simulink model "sst_cllc_ttype_inv_discrete"  (R2026b)
settings: Solver=ode23tb  StopTime=simlength  FixedStep=tc  MaxStep=glb_time.tc
values from neighbouring files (symbols this model uses):
  param = sst_cllc_ttype_setup(param)    [init_model.m]
undefined symbols (not defined in the file or in its folder): afe_ctrl, glb_time, grid_emu, hwdata, omega_set, single_phase_inverter_ctrl, sst_num_of_modules
libraries: fl_lib x28, nesl_utility x16, discrete_time_low_pass_filter x4, lithium_ion_battery x2, cllc_dcx x2, dclink_for_three_levels x2, full_bridge_three_level_ttype_ideal_switch_based_model x2, full_bridge_three_level_ttype_mosfet_based_model x2, simulink x2, cstblocks_lti x2, single_phase_three_levels_PWM_modulator x2, dq_vector_pi x2
(part 3 of 3)

== system sst_cllc_ttype_inv_discrete/single_phase_inverter_modA/single phase inverter control/single_phase_inverter_ctrl/single_phase_pll/pi-ctrl ==
  x : Inport
  xref : Inport  Port=2
  1/Ti : Gain  Gain=kp  SaturateOnIntegerOverflow=on  OutDataTypeStr=Inherit: Same as input  ParamDataTypeStr=Inherit: Same as input
  Saturation : Saturate  UpperLimit=sat_pos  LowerLimit=sat_neg
  Sum1 : Sum  Inputs=+++  SaturateOnIntegerOverflow=on
  Sum2 : Sum  Inputs=-+  SaturateOnIntegerOverflow=on
  Sum3 : Sum  Inputs=-+  SaturateOnIntegerOverflow=on
  Unit Delay4 : UnitDelay  SampleTime=-1
  kp : Gain  Gain=ki*ts  SaturateOnIntegerOverflow=on  OutDataTypeStr=Inherit: Same as input  ParamDataTypeStr=Inherit: Same as input
  u : Outport
  wires:
  Saturation/1 -> Sum3/2, u/1
  Unit Delay4/1 -> Sum1/3
  Sum1/1 -> Saturation/1
  Sum3/1 -> Unit Delay4/1
  1/Ti/1 -> Sum3/1, Sum1/1
  Sum2/1 -> 1/Ti/1, kp/1
  kp/1 -> Sum1/2
  x/1 -> Sum2/1
  xref/1 -> Sum2/2

== system sst_cllc_ttype_inv_discrete/single_phase_inverter_modB/single phase inverter control/single_phase_inverter_ctrl/single_phase_current_control/current_reference_generation ==
  mag_ref : Inport
  phase : Inport  Port=2
  Bus Creator : BusCreator  Inputs=2
  Product : Product
  Product1 : Product
  Sin : Trigonometry  Operator=cos
  Sin1 : Trigonometry
  is_ref : Outport
  id_ref : Outport  Port=2
  wires:
  Bus Creator/1 -> is_ref/1
  Product1/1 -> Bus Creator/2  "is_ref_beta"
  Product/1 -> Bus Creator/1  "is_ref_alpha"
  Sin1/1 -> Product1/2
  mag_ref/1 -> Product/1, Product1/1, id_ref/1
  phase/1 -> Sin/1, Sin1/1
  Sin/1 -> Product/2

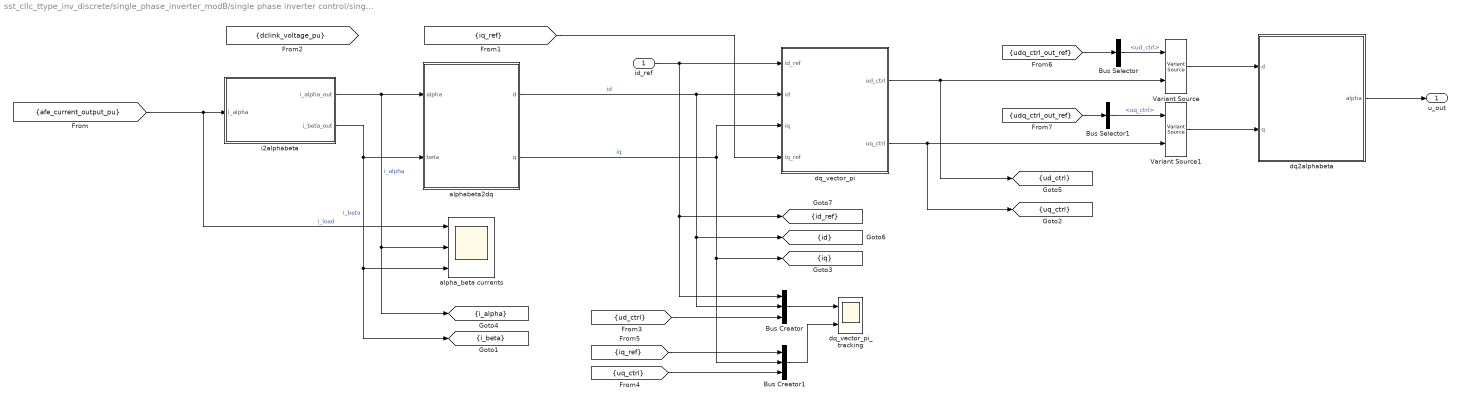
== system sst_cllc_ttype_inv_discrete/single_phase_inverter_modB/single phase inverter control/single_phase_inverter_ctrl/single_phase_current_control/dqpi_current_controller ==
  id_ref : Inport
  Bus Creator : BusCreator  Inputs=3
  Bus Creator1 : BusCreator  Inputs=3
  Bus Selector : BusSelector  OutputSignals=ud_ctrl
  Bus Selector1 : BusSelector  OutputSignals=uq_ctrl
  Variant Source : VariantSource  VariantControls={true, false}
  Variant Source1 : VariantSource  VariantControls={true, false}
  alpha_beta currents : Scope  NumInputPorts=3
      settings: ActiveDisplayYMinimum=-43.020049026506776  ActiveDisplayYMaximum=15.212667801061009  DataLoggingVariableName=ScopeData2
  alphabeta2dq : Subsystem
  dq2alphabeta : Subsystem
  dq_vector_pi : Subsystem
  dq_vector_pi_tracking : Scope  NumInputPorts=2
      settings: ActiveDisplayYMinimum=-5.8450231123834442  ActiveDisplayYMaximum=20.947282871449747  DataLoggingVariableName=ScopeData8
  i2alphabeta : Subsystem
  u_out : Outport
  tag scope: i_alpha=scoped, i_beta=scoped, id=scoped, id_ref=scoped, iq=scoped, ud_ctrl=scoped, uq_ctrl=scoped
  wires:
  dq_vector_pi/1(ud_ctrl) -> [ud_ctrl], Variant Source/2
  i2alphabeta/2(i_beta_out) -> alphabeta2dq/2(beta), alpha_beta currents/3, [i_beta]  "i_beta"
  i2alphabeta/1(i_alpha_out) -> alphabeta2dq/1(alpha), [i_alpha], alpha_beta currents/2  "i_alpha"
  [afe_current_output_pu] -> i2alphabeta/1(i_alpha), alpha_beta currents/1  "i_load"
  [iq_ref] -> Bus Creator1/1
  [uq_ctrl] -> Bus Creator1/3
  [ud_ctrl] -> Bus Creator/3
  Bus Creator/1 -> dq_vector_pi_tracking/1
  Bus Creator1/1 -> dq_vector_pi_tracking/2
  [iq_ref] -> dq_vector_pi/4(iq_ref)
  alphabeta2dq/2("q ") -> [iq], Bus Creator1/2, dq_vector_pi/3(iq)  "iq"
  alphabeta2dq/1("d ") -> dq_vector_pi/2(id), [id], Bus Creator/2  "id"
  id_ref/1 -> [id_ref], Bus Creator/1, dq_vector_pi/1(id_ref)
  dq2alphabeta/1(alpha) -> u_out/1
  [udq_ctrl_out_ref] -> Bus Selector/1
  Variant Source/1 -> dq2alphabeta/1(d)
  Bus Selector/1 -> Variant Source/1  "<ud_ctrl>"
  Bus Selector1/1 -> Variant Source1/1  "<uq_ctrl>"
  [udq_ctrl_out_ref] -> Bus Selector1/1
  dq_vector_pi/2(uq_ctrl) -> Variant Source1/2, [uq_ctrl]
  Variant Source1/1 -> dq2alphabeta/2(q)

== system sst_cllc_ttype_inv_discrete/single_phase_inverter_modB/single phase inverter control/single_phase_inverter_ctrl/single_phase_pll/double_integrator_observer ==
  theta : Inport
  Gain : Gain  Gain=afe_ctrl.di_obs.Ldso  Multiplication=Matrix(K*u)
  Gain1 : Gain  Gain=afe_ctrl.di_obs.Adso  Multiplication=Matrix(K*u)
  Gain2 : Gain  Gain=afe_ctrl.di_obs.Cso  Multiplication=Matrix(K*u)
  Selector : Selector  InputPortWidth=2  IndexOptions=Index vector (dialog)  Indices=2  OutputSizes=1  RuntimeRangeChecks=off
  Sum : Sum  Inputs=-+|
  Sum1 : Sum  Inputs=|++
  Unit Delay : UnitDelay  SampleTime=-1
  bounder1 : MATLAB Function  TreatAsAtomicUnit=on
  bounder2 : MATLAB Function  TreatAsAtomicUnit=on
  kp3 : Gain  Gain=1/grid_emu.omega_grid_nom  SaturateOnIntegerOverflow=on  OutDataTypeStr=Inherit: Same as input  ParamDataTypeStr=Inherit: Same as input
  phase_hat : Outport
  omega_hat : Outport  Port=2
  wires:
  kp3/1 -> omega_hat/1
  Selector/1 -> kp3/1
  bounder2/1(y) -> Sum/1, phase_hat/1  "theta_hat_bounded"
  bounder1/1(y) -> Gain/1  "e_bounded"
  theta/1 -> Sum/2  "theta"
  Unit Delay/1 -> Gain2/1, Gain1/1, Selector/1
  Sum/1 -> bounder1/1(u)  "e"
  Sum1/1 -> Unit Delay/1
  Gain1/1 -> Sum1/2
  Gain2/1 -> bounder2/1(u)  "theta_hat"
  Gain/1 -> Sum1/1

== system sst_cllc_ttype_inv_discrete/single_phase_inverter_modB/single phase inverter control/single_phase_inverter_ctrl/single_phase_pll/pi-ctrl ==
  x : Inport
  xref : Inport  Port=2
  1/Ti : Gain  Gain=kp  SaturateOnIntegerOverflow=on  OutDataTypeStr=Inherit: Same as input  ParamDataTypeStr=Inherit: Same as input
  Saturation : Saturate  UpperLimit=sat_pos  LowerLimit=sat_neg
  Sum1 : Sum  Inputs=+++  SaturateOnIntegerOverflow=on
  Sum2 : Sum  Inputs=-+  SaturateOnIntegerOverflow=on
  Sum3 : Sum  Inputs=-+  SaturateOnIntegerOverflow=on
  Unit Delay4 : UnitDelay  SampleTime=-1
  kp : Gain  Gain=ki*ts  SaturateOnIntegerOverflow=on  OutDataTypeStr=Inherit: Same as input  ParamDataTypeStr=Inherit: Same as input
  u : Outport
  wires:
  xref/1 -> Sum2/2
  x/1 -> Sum2/1
  kp/1 -> Sum1/2
  Sum2/1 -> kp/1, 1/Ti/1
  1/Ti/1 -> Sum1/1, Sum3/1
  Sum3/1 -> Unit Delay4/1
  Sum1/1 -> Saturation/1
  Unit Delay4/1 -> Sum1/3
  Saturation/1 -> u/1, Sum3/2

== system sst_cllc_ttype_inv_discrete/single_phase_inverter_modA/single phase inverter control/single_phase_inverter_ctrl/single_phase_current_control/dqpi_current_controller/alphabeta2dq ==
  alpha : Inport
  beta : Inport  Port=2
  MATLAB Function : MATLAB Function  TreatAsAtomicUnit=on
  "d " : Outport  VectorParamsAs1DForOutWhenUnconnected=off
  "q " : Outport  Port=2  VectorParamsAs1DForOutWhenUnconnected=off
  wires:
  alpha/1 -> MATLAB Function/1(alpha)
  beta/1 -> MATLAB Function/2(beta)
  MATLAB Function/1(d) -> "d "/1
  MATLAB Function/2(q) -> "q "/1
  [phase_grid] -> MATLAB Function/3(phase)

== system sst_cllc_ttype_inv_discrete/single_phase_inverter_modA/single phase inverter control/single_phase_inverter_ctrl/single_phase_current_control/dqpi_current_controller/dq2alphabeta ==
  d : Inport
  q : Inport  Port=2
  MATLAB Function : MATLAB Function  TreatAsAtomicUnit=on
  alpha : Outport  VectorParamsAs1DForOutWhenUnconnected=off
  wires:
  d/1 -> MATLAB Function/1(d)
  q/1 -> MATLAB Function/2(q)
  MATLAB Function/1(alpha) -> alpha/1
  [phase_grid] -> MATLAB Function/3(phase)

== system sst_cllc_ttype_inv_discrete/single_phase_inverter_modA/single phase inverter control/single_phase_inverter_ctrl/single_phase_current_control/dqpi_current_controller/dq_vector_pi ==
  id_ref : Inport
  id : Inport  Port=2
  iq : Inport  Port=3
  iq_ref : Inport  Port=4
  dq_vector_pi : dq_vector_pi/dq_vector_pi  kp=single_phase_inverter_ctrl.kp_inv  ki=single_phase_inverter_ctrl.ki_inv  ts=glb_time.ts_inv  lim_ctrl_out=single_phase_inverter_ctrl.u_lim  CTRPIFF_CLIP_RELEASE=CTRPIFF_CLIP_RELEASE
  ud_ctrl : Outport
  uq_ctrl : Outport  Port=2
  wires:
  id_ref/1 -> dq_vector_pi/1  "id_ref"
  iq_ref/1 -> dq_vector_pi/3  "iq_ref"
  dq_vector_pi/1 -> ud_ctrl/1  "ud_ctrl"
  iq/1 -> dq_vector_pi/4  "iq"
  id/1 -> dq_vector_pi/2  "id"
  dq_vector_pi/2 -> uq_ctrl/1  "uq_ctrl"
  [dclink_voltage_pu] -> dq_vector_pi/5

== system sst_cllc_ttype_inv_discrete/single_phase_inverter_modA/single phase inverter control/single_phase_inverter_ctrl/single_phase_current_control/dqpi_current_controller/i2alphabeta ==
  i_alpha : Inport
  FHTalpha : Subsystem
  i_alpha_out : Outport
  i_beta_out : Outport  Port=2
  wires:
  i_alpha/1 -> FHTalpha/1(u)
  FHTalpha/1(ualpha) -> i_alpha_out/1  "u_fht_alpha"
  FHTalpha/2(ubeta) -> i_beta_out/1  "v_fht_alpha"

== system sst_cllc_ttype_inv_discrete/single_phase_inverter_modB/single phase inverter control/single_phase_inverter_ctrl/single_phase_current_control/dqpi_current_controller/alphabeta2dq ==
  alpha : Inport
  beta : Inport  Port=2
  MATLAB Function : MATLAB Function  TreatAsAtomicUnit=on
  "d " : Outport  VectorParamsAs1DForOutWhenUnconnected=off
  "q " : Outport  Port=2  VectorParamsAs1DForOutWhenUnconnected=off
  wires:
  [phase_grid] -> MATLAB Function/3(phase)
  MATLAB Function/2(q) -> "q "/1
  MATLAB Function/1(d) -> "d "/1
  beta/1 -> MATLAB Function/2(beta)
  alpha/1 -> MATLAB Function/1(alpha)

== system sst_cllc_ttype_inv_discrete/single_phase_inverter_modB/single phase inverter control/single_phase_inverter_ctrl/single_phase_current_control/dqpi_current_controller/dq2alphabeta ==
  d : Inport
  q : Inport  Port=2
  MATLAB Function : MATLAB Function  TreatAsAtomicUnit=on
  alpha : Outport  VectorParamsAs1DForOutWhenUnconnected=off
  wires:
  [phase_grid] -> MATLAB Function/3(phase)
  MATLAB Function/1(alpha) -> alpha/1
  q/1 -> MATLAB Function/2(q)
  d/1 -> MATLAB Function/1(d)

== system sst_cllc_ttype_inv_discrete/single_phase_inverter_modB/single phase inverter control/single_phase_inverter_ctrl/single_phase_current_control/dqpi_current_controller/dq_vector_pi ==
  id_ref : Inport
  id : Inport  Port=2
  iq : Inport  Port=3
  iq_ref : Inport  Port=4
  dq_vector_pi : dq_vector_pi/dq_vector_pi  kp=single_phase_inverter_ctrl.kp_inv  ki=single_phase_inverter_ctrl.ki_inv  ts=glb_time.ts_inv  lim_ctrl_out=single_phase_inverter_ctrl.u_lim  CTRPIFF_CLIP_RELEASE=CTRPIFF_CLIP_RELEASE
  ud_ctrl : Outport
  uq_ctrl : Outport  Port=2
  wires:
  [dclink_voltage_pu] -> dq_vector_pi/5
  dq_vector_pi/2 -> uq_ctrl/1  "uq_ctrl"
  id/1 -> dq_vector_pi/2  "id"
  iq/1 -> dq_vector_pi/4  "iq"
  dq_vector_pi/1 -> ud_ctrl/1  "ud_ctrl"
  iq_ref/1 -> dq_vector_pi/3  "iq_ref"
  id_ref/1 -> dq_vector_pi/1  "id_ref"

== system sst_cllc_ttype_inv_discrete/single_phase_inverter_modB/single phase inverter control/single_phase_inverter_ctrl/single_phase_current_control/dqpi_current_controller/i2alphabeta ==
  i_alpha : Inport
  FHTalpha : Subsystem
  i_alpha_out : Outport
  i_beta_out : Outport  Port=2
  wires:
  FHTalpha/2(ubeta) -> i_beta_out/1  "v_fht_alpha"
  FHTalpha/1(ualpha) -> i_alpha_out/1  "u_fht_alpha"
  i_alpha/1 -> FHTalpha/1(u)

== system sst_cllc_ttype_inv_discrete/single_phase_inverter_modA/single phase inverter control/single_phase_inverter_ctrl/single_phase_current_control/dqpi_current_controller/i2alphabeta/FHTalpha ==
  u : Inport
  Gain : Gain  Gain=single_phase_inverter_ctrl.fht_load.Ld_fht  Multiplication=Matrix(K*u)
  Gain1 : Gain  Gain=single_phase_inverter_ctrl.fht_load.Ad_fht  Multiplication=Matrix(K*u)
  Gain2 : Gain  Gain=single_phase_inverter_ctrl.fht_load.Cfht  Multiplication=Matrix(K*u)
  Gain3 : Gain  Gain=-1/single_phase_inverter_ctrl.omega_base
  Selector : Selector  InputPortWidth=2  IndexOptions=Index vector (dialog)  Indices=1  OutputSizes=1  RuntimeRangeChecks=off
  Selector1 : Selector  InputPortWidth=2  IndexOptions=Index vector (dialog)  Indices=2  OutputSizes=1  RuntimeRangeChecks=off
  Sum : Sum  Inputs=-+|
  Sum1 : Sum  Inputs=|++
  Unit Delay : UnitDelay  SampleTime=-1
  ualpha : Outport
  ubeta : Outport  Port=2
  wires:
  u/1 -> Sum/2
  Unit Delay/1 -> Gain2/1, Selector1/1, Selector/1, Gain1/1
  Sum/1 -> Gain/1
  Sum1/1 -> Unit Delay/1
  Gain1/1 -> Sum1/2
  Gain2/1 -> Sum/1
  Selector/1 -> ualpha/1
  Gain/1 -> Sum1/1
  Selector1/1 -> Gain3/1
  Gain3/1 -> ubeta/1

== system sst_cllc_ttype_inv_discrete/single_phase_inverter_modB/single phase inverter control/single_phase_inverter_ctrl/single_phase_current_control/dqpi_current_controller/i2alphabeta/FHTalpha ==
  u : Inport
  Gain : Gain  Gain=single_phase_inverter_ctrl.fht_load.Ld_fht  Multiplication=Matrix(K*u)
  Gain1 : Gain  Gain=single_phase_inverter_ctrl.fht_load.Ad_fht  Multiplication=Matrix(K*u)
  Gain2 : Gain  Gain=single_phase_inverter_ctrl.fht_load.Cfht  Multiplication=Matrix(K*u)
  Gain3 : Gain  Gain=-1/single_phase_inverter_ctrl.omega_base
  Selector : Selector  InputPortWidth=2  IndexOptions=Index vector (dialog)  Indices=1  OutputSizes=1  RuntimeRangeChecks=off
  Selector1 : Selector  InputPortWidth=2  IndexOptions=Index vector (dialog)  Indices=2  OutputSizes=1  RuntimeRangeChecks=off
  Sum : Sum  Inputs=-+|
  Sum1 : Sum  Inputs=|++
  Unit Delay : UnitDelay  SampleTime=-1
  ualpha : Outport
  ubeta : Outport  Port=2
  wires:
  Gain3/1 -> ubeta/1
  Selector1/1 -> Gain3/1
  Gain/1 -> Sum1/1
  Selector/1 -> ualpha/1
  Gain2/1 -> Sum/1
  Gain1/1 -> Sum1/2
  Sum1/1 -> Unit Delay/1
  Sum/1 -> Gain/1
  Unit Delay/1 -> Gain1/1, Selector/1, Selector1/1, Gain2/1
  u/1 -> Sum/2

== matlab function sst_cllc_ttype_inv_discrete/single_phase_inverter_modB/single phase inverter control/single_phase_inverter_ctrl/single_phase_pll/alphabeta2xieta ==
  data: alpha input; xi output; beta input; gamma input; eta output
function [xi,eta] = alphabeta2xieta(alpha,beta,gamma)
    xi  =  alpha*cos(gamma) + beta*sin(gamma);
    eta = -alpha*sin(gamma) + beta*cos(gamma);
end

== matlab function sst_cllc_ttype_inv_discrete/single_phase_inverter_modB/single phase inverter control/single_phase_inverter_ctrl/single_phase_pll/bounder2 ==
  data: u input; y output
function y = bounder(u)
    
    y = -pi + mod(u+3*pi,2*pi);
   
end

== matlab function sst_cllc_ttype_inv_discrete/single_phase_inverter_modB/single phase inverter control/single_phase_inverter_ctrl/single_phase_pll/double_integrator_observer/bounder1 ==
  data: u input; y output
function y = bounder(u)
    
    y = -pi + mod(u+3*pi,2*pi);
   
end

== matlab function sst_cllc_ttype_inv_discrete/single_phase_inverter_modB/single phase inverter control/single_phase_inverter_ctrl/single_phase_pll/double_integrator_observer/bounder2 ==
  data: u input; y output
function y = bounder(u)
    
    y = -pi + mod(u+3*pi,2*pi);
   
end

== matlab function sst_cllc_ttype_inv_discrete/single_phase_inverter_modB/single phase inverter control/single_phase_inverter_ctrl/single_phase_pll/xieta2alphabeta ==
  data: xi input; alpha output; eta input; gamma input; beta output
function [alpha,beta] = xieta2alphabeta(xi,eta,gamma)
    alpha  = xi*cos(gamma) - eta*sin(gamma);
    beta = xi*sin(gamma) + eta*cos(gamma);
end

== matlab function sst_cllc_ttype_inv_discrete/single_phase_inverter_modA/single phase inverter control/single_phase_inverter_ctrl/single_phase_pll/double_integrator_observer/bounder1 ==
  data: u input; y output
function y = bounder(u)
    
    y = -pi + mod(u+3*pi,2*pi);
   
end

== matlab function sst_cllc_ttype_inv_discrete/single_phase_inverter_modA/single phase inverter control/single_phase_inverter_ctrl/single_phase_pll/double_integrator_observer/bounder2 ==
  data: u input; y output
function y = bounder(u)
    
    y = -pi + mod(u+3*pi,2*pi);
   
end

== matlab function sst_cllc_ttype_inv_discrete/single_phase_inverter_modA/single phase inverter control/single_phase_inverter_ctrl/single_phase_pll/xieta2alphabeta ==
  data: xi input; alpha output; eta input; gamma input; beta output
function [alpha,beta] = xieta2alphabeta(xi,eta,gamma)
    alpha  = xi*cos(gamma) - eta*sin(gamma);
    beta = xi*sin(gamma) + eta*cos(gamma);
end

== matlab function sst_cllc_ttype_inv_discrete/line_source/phase_gen/bounder1 ==
  data: u input; y output
function y = bounder(u)
    
    y = -pi + mod(u+3*pi,2*pi);
end

== matlab function sst_cllc_ttype_inv_discrete/single_phase_inverter_modA/single phase inverter control/single_phase_inverter_ctrl/single_phase_pll/alphabeta2xieta ==
  data: alpha input; xi output; beta input; gamma input; eta output
function [xi,eta] = alphabeta2xieta(alpha,beta,gamma)
    xi  =  alpha*cos(gamma) + beta*sin(gamma);
    eta = -alpha*sin(gamma) + beta*cos(gamma);
end

== matlab function sst_cllc_ttype_inv_discrete/single_phase_inverter_modB/single phase inverter control/single_phase_inverter_ctrl/single_phase_current_control/dqpi_current_controller/alphabeta2dq/MATLAB Function ==
  data: alpha input; d output; beta input; phase input; q output
function [d, q] = alphabeta2dq(alpha, beta, phase)

d = alpha*cos(phase) + beta*sin(phase);
q = -alpha*sin(phase) + beta*cos(phase);

== matlab function sst_cllc_ttype_inv_discrete/single_phase_inverter_modA/single phase inverter control/single_phase_inverter_ctrl/single_phase_pll/bounder2 ==
  data: u input; y output
function y = bounder(u)
    
    y = -pi + mod(u+3*pi,2*pi);
   
end

== matlab function sst_cllc_ttype_inv_discrete/single_phase_inverter_modB/single phase inverter control/single_phase_inverter_ctrl/single_phase_current_control/dqpi_current_controller/dq2alphabeta/MATLAB Function ==
  data: d input; alpha output; q input; phase input; beta output
function [alpha, beta] = dq2alphabeta(d, q, phase)

alpha = d*cos(phase) - q*sin(phase);
beta = d*sin(phase) + q*cos(phase);

== matlab function sst_cllc_ttype_inv_discrete/single_phase_inverter_modA/single phase inverter control/single_phase_inverter_ctrl/single_phase_current_control/dqpi_current_controller/alphabeta2dq/MATLAB Function ==
  data: alpha input; d output; beta input; phase input; q output
function [d, q] = alphabeta2dq(alpha, beta, phase)

d = alpha*cos(phase) + beta*sin(phase);
q = -alpha*sin(phase) + beta*cos(phase);

== matlab function sst_cllc_ttype_inv_discrete/single_phase_inverter_modA/single phase inverter control/single_phase_inverter_ctrl/single_phase_current_control/dqpi_current_controller/dq2alphabeta/MATLAB Function ==
  data: d input; alpha output; q input; phase input; beta output
function [alpha, beta] = dq2alphabeta(d, q, phase)

alpha = d*cos(phase) - q*sin(phase);
beta = d*sin(phase) + q*cos(phase);
